simulink model "NEPTUN_ZH_Z5"  (R2026a)
settings: Solver=ode45  StopTime=10e-3  MaxStep=25e-6/25  EnableMultiTasking=on
libraries: NEPTUN_MK x1
settings Model: Creator=oktato  LastModifiedBy=Szalay
settings HardwareCC: ProdHWDeviceType=32-bit Generic

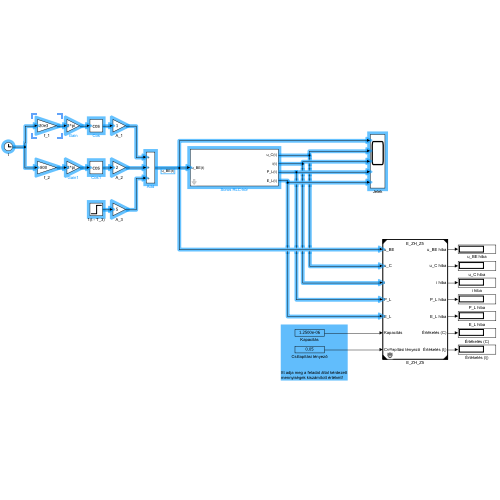
[thumbnail: Simulink's stored preview of the top-level diagram]
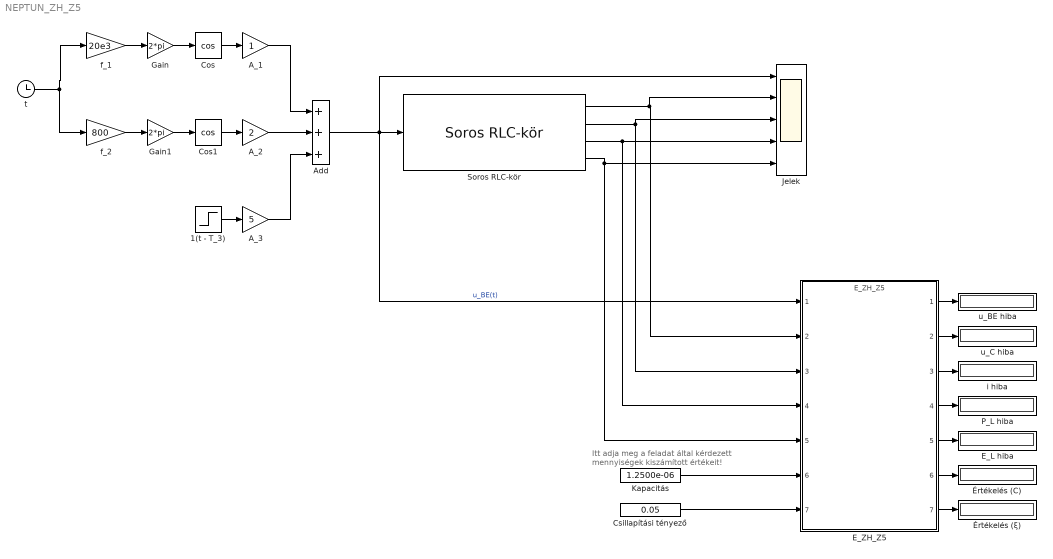
== system NEPTUN_ZH_Z5 ==
  note: Itt adja meg a feladat által kérdezett
      | mennyiségek kiszámított értékeit!
  1(t - T_3) : Step  Time=5e-3  SampleTime=0
  A_1 : Gain
  A_2 : Gain  Gain=2
  A_3 : Gain  Gain=5
  Add : Sum  Inputs=+++
  Cos : Trigonometry  Operator=cos
  Cos1 : Trigonometry  Operator=cos
  Csillapítási tényező : Constant  Value=0.05
  E_L hiba : Display
  E_ZH_Z5 : ModelReference  ModelNameDialog=E_ZH_Z5.slxp  ModelReferenceVersion=3.7  CopyOfModelProtected=on
  Gain : Gain  Gain=2*pi
  Gain1 : Gain  Gain=2*pi
  Jelek : Scope  NumInputPorts=5
      settings: ActiveDisplayYMinimum=-4.3748123260415985  ActiveDisplayYMaximum=9.3749791473379549
  Kapacitás : Constant  Value=1.2500e-06
  P_L hiba : Display
  Soros RLC-kör : NEPTUN_MK/Soros RLC-kör  R=2  L=500e-6  tau=25e-6  i_0=-200e-3  u_C0=1
  f_1 : Gain  Gain=20e3
  f_2 : Gain  Gain=800
  i hiba : Display
  t : Clock
  u_BE hiba : Display
  u_C hiba : Display
  Értékelés (C) : Display
  Értékelés (ξ) : Display
  wires:
  E_ZH_Z5/3 -> i hiba/1
  E_ZH_Z5/1 -> u_BE hiba/1
  E_ZH_Z5/2 -> u_C hiba/1
  Kapacitás/1 -> E_ZH_Z5/6
  Csillapítási tényező/1 -> E_ZH_Z5/7
  E_ZH_Z5/7 -> Értékelés (ξ)/1
  E_ZH_Z5/6 -> Értékelés (C)/1
  E_ZH_Z5/4 -> P_L hiba/1
  E_ZH_Z5/5 -> E_L hiba/1
  Add/1 -> Jelek/1, E_ZH_Z5/1, Soros RLC-kör/1  "u_BE(t)"
  A_1/1 -> Add/1
  A_2/1 -> Add/2
  A_3/1 -> Add/3
  Cos/1 -> A_1/1
  Cos1/1 -> A_2/1
  1(t - T_3)/1 -> A_3/1
  Gain/1 -> Cos/1
  Gain1/1 -> Cos1/1
  f_1/1 -> Gain/1
  f_2/1 -> Gain1/1
  t/1 -> f_1/1, f_2/1
  Soros RLC-kör/1 -> Jelek/2, E_ZH_Z5/2
  Soros RLC-kör/2 -> E_ZH_Z5/3, Jelek/3
  Soros RLC-kör/3 -> E_ZH_Z5/4, Jelek/4
  Soros RLC-kör/4 -> Jelek/5, E_ZH_Z5/5
